simulink model "R4_ArduPilot_JSON"  (R2025b)
settings: Solver=ode4  StartTime=0.0  StopTime=P.stopTime  FixedStep=P.dt  RelTol=1e-3
InitFcn:
  | ww=get_param('R4_ArduPilot_JSON','ModelWorkspace'); pp=getVariable(ww,'P'); assignin(ww,'V',[pp.configurationCode(:);pp.mass(:);pp.cg(:);pp.inertia(:);pp.massCtrl(:);pp.cgCtrl(:);pp.inertiaCtrl(:);pp.g(:);pp.dt(:);pp.Ts(:);pp.stopTime(:);pp.sensorDelaySamples(:);pp.seed(:);pp.noiseScale(:);pp.sensorStd(:);pp.jetRadius(:);pp.motorRadius(:);pp.jetArea(:);pp.vaneArea(:);pp.vaneRadius(:);pp.forceZ(:);pp.hingeZ(:);pp.Lctrl(:);pp.CLalpha(:);pp.CLalphaCtrl(:);pp.stallAngle(:);pp.stallAngleCtrl(:);pp.effectiveness(:);pp.effectivenessCtrl(:);pp.CD0(:);pp.inducedDragK(:);pp.deltaMax(:);pp.servoRate(:);pp.servoTau(:);pp.fanTau(:);pp.fanTauCtrl(:);pp.TmaxNominal(:);pp.thrustScale(:);pp.voltageFinalScale(:);pp.voltageStart(:);pp.voltageRamp(:);pp.residualTorquePerN(:);pp.residualTorqueCtrl(:);pp.angularDrag(:);pp.linearDrag(:);pp.quadraticDrag(:);pp.angleGain(:);pp.rateKp(:);pp.rateKi(:);pp.rateLimit(:);pp.torqueIlimit(:);pp.altKp(:);pp.altKd(:);pp.altKi(:);pp.forceIlimit(:);pp.positionEnabled(:);pp.positionKp(:);pp.positionKd(:);pp.positionTiltLimit(:);pp.awTorque(:);pp.awForce(:);pp.controlEnabled(:);pp.scenario(:);pp.zReference(:);pp.initialEuler(:);pp.initialPosition(:);pp.initialVelocity(:);pp.forceDisturbance(:);pp.torqueDisturbance(:);pp.pulseTimes(:);pp.tetherEnabled(:);pp.groundEnabled(:);pp.tetherStiffness(:);pp.tetherDamping(:);pp.upperLength(:);pp.lowerLength(:);pp.groundStiffness(:);pp.groundDamping(:);pp.groundFriction(:);pp.controllerVersion(:);pp.heightPositionKp(:);pp.verticalSpeedKp(:);pp.verticalSpeedKi(:);pp.verticalSpeedLimit(:);pp.verticalAccelLimit(:);pp.throttleExpo(:);pp.startupEnabled(:);pp.startupSpoolBegin(:);pp.startupSpoolEnd(:);pp.startupRampNps(:);pp.startupMaxThrustFactor(:);pp.startupTimeout(:);pp.liftDetectHeight(:);pp.liftDetectDuration(:);pp.startupAbortTilt(:);pp.referenceGovernor(:);pp.tetherHeightLimit(:);pp.referenceStart(:);pp.referenceRiseTime(:);pp.referenceAngleStep(:);pp.referenceStepBegin(:);pp.referenceStepEnd(:);pp.staticTrimEnabled(:);pp.accelerationFilterTau(:);pp.eyeBody(:);pp.upperAnchor(:);pp.lowerAnchor(:);pp.feetBody(:);pp.floorZ(:);pp.trimT(:);pp.trimTau(:);pp.trimDelta(:);pp.x0(:);pp.y0(:);pp.trimWrench(:);pp.linkTs(:);pp.rangeNoiseStd(:);pp.rangeBias(:);pp.rangeSensorBodyZ(:);pp.rngSeed(:);pp.windWorld(:);pp.jsonPort(:)]); clear ww pp;
model workspace (MAT data in the model file):
  P.configurationCode = 5
  P.mass = 2.0128
  P.cg = [-0.00056; 0.00028; 0.31804]
  P.inertia = [0.042126; 0.042115; 0.007025]
  P.massCtrl = 2.0128
  P.cgCtrl = [-0.00056; 0.00028; 0.31804]
  P.inertiaCtrl = [0.042126; 0.042115; 0.007025]
  P.g = 9.80665
  P.dt = 0.000416666666667
  P.Ts = 0.005
  P.stopTime = 300
  P.sensorDelaySamples = 2
  P.seed = 41
  P.noiseScale = 1
  P.sensorStd = [0.001; 0.001; 0.001; 0.005; 0.005; 0.005; 0.00174532925199; 0.00174532925199; 0.00174532925199; 0.00349065850399; 0.00349065850399; 0.00349065850399; 0.05]
  P.jetRadius = 0.04
  P.motorRadius = 0.016
  P.jetArea = 0.00422230052642
  P.vaneArea = 0.000576
  P.vaneRadius = 0.031
  P.forceZ = 0.1316
  P.hingeZ = 0.13
  P.Lctrl = 0.18644
  P.CLalpha = 1.3
  P.CLalphaCtrl = 1.3
  P.stallAngle = 0.436332312999
  P.stallAngleCtrl = 0.436332312999
  P.effectiveness = 1
  P.effectivenessCtrl = 1
  P.CD0 = 0.015
  P.inducedDragK = 0.707355302631
  P.deltaMax = 0.349065850399
  P.servoRate = 12.3199711905
  P.servoTau = 0.03
  P.fanTau = 0.15
  P.fanTauCtrl = 0.15
  P.TmaxNominal = 27.6155264
  P.thrustScale = 1
  P.voltageFinalScale = 1
  P.voltageStart = 6
  P.voltageRamp = 1
  P.residualTorquePerN = 0.001
  P.residualTorqueCtrl = 0.001
  P.angularDrag = [0.002; 0.002; 0.001]
  P.linearDrag = [0.15; 0.15; 0.08]
  P.quadraticDrag = [0.08; 0.08; 0.05]
  P.angleGain = [2; 2; 1.8]
  P.rateKp = [0.32; 0.32; 0.08]
  P.rateKi = [0.35; 0.35; 0.08]
  P.rateLimit = [0.7; 0.7; 0.8]
  P.torqueIlimit = [0.15; 0.15; 0.06]
  P.altKp = 4
  P.altKd = 3.5
  P.altKi = 3
  P.forceIlimit = 8
  P.positionEnabled = 0
  P.positionKp = 0.6
  P.positionKd = 1.4
  P.positionTiltLimit = 0.13962634016
  P.awTorque = 6
  P.awForce = 2
  P.controlEnabled = 1
  P.scenario = 1
  P.zReference = 5
  P.initialEuler = [0; 0; 0]
  P.initialPosition = [0; 0; 0]
  P.initialVelocity = [0; 0; 0]
  P.forceDisturbance = [0  0; 0  0; 0  0]
  P.torqueDisturbance = [0  0; 0  0; 0  0]
  P.pulseTimes = [95  95.2; 105  105.5]
  P.tetherEnabled = 0
  P.groundEnabled = 1
  P.tetherStiffness = 5000
  P.tetherDamping = 35
  P.upperLength = 0.424
  P.lowerLength = 0.575
  P.groundStiffness = 8000
  P.groundDamping = 50
  P.groundFriction = 0.4
  P.controllerVersion = 2
  P.heightPositionKp = 1.2
  P.verticalSpeedKp = 6
  P.verticalSpeedKi = 2.5
  P.verticalSpeedLimit = 0.15
  P.verticalAccelLimit = 3
  P.throttleExpo = 0.6
  P.startupEnabled = 1
  P.startupSpoolBegin = 0.5
  P.startupSpoolEnd = 2
  P.startupRampNps = 1.2
  P.startupMaxThrustFactor = 1.32
  P.startupTimeout = 14
  P.liftDetectHeight = 0.008
  P.liftDetectDuration = 0.05
  P.startupAbortTilt = 0.349065850399
  P.referenceGovernor = 1
  P.tetherHeightLimit = 0.075
  P.referenceStart = 2
  P.referenceRiseTime = 4
  P.referenceAngleStep = [0; 0; 0]
  P.referenceStepBegin = 9
  P.referenceStepEnd = 12
  P.staticTrimEnabled = 1
  P.accelerationFilterTau = 0.1
  P.eyeBody = [0.0698564645563  -0.0687364645563  -0.0687364645563  0.0698564645563; 0.0690164645563  0.0690164645563  -0.0695764645563  -0.0695764645563; 0.11946  0.11946  0.11946  0.11946]
  P.upperAnchor = [0.270674790413  -0.269554790413  -0.269554790413  0.270674790413; 0.269834790413  0.269834790413  -0.270394790413  -0.270394790413; 0.43396  0.43396  0.43396  0.43396]
  P.lowerAnchor = [0.25056  -0.24944  -0.24944  0.25056; 0.16472  0.16472  -0.16528  -0.16528; -0.31804  -0.31804  -0.31804  -0.31804]
  P.feetBody = [0.163194559673  -0.162074559673  -0.162074559673  0.163194559673; 0.162354559673  0.162354559673  -0.162914559673  -0.162914559673; -0.33304  -0.33304  -0.33304  -0.33304]
  P.floorZ = -0.33304
  P.trimT = 19.8749456665
  P.trimTau = [0.00556498478663; 0.0111299695733; -0.0198749456665]
  P.trimDelta = [-0.0825320279718; -0.0740418704167; -0.099550958918; -0.108087721792]
  P.x0 = [0; 0; 0; 0; 0; 0; 1; 0; 0; 0; 0; 0; 0; 0; 0; 0; 0; 0]
  P.y0 = [0; 0; 0; 0; 0; 0; 0; 0; 0; 0; 0; 0; 0]
  P.trimWrench = [19.8749456665; 0.00556498478663; 0.0111299695733; -0.0198749456665]
  P.linkTs = 0.000833333333333
  P.rangeNoiseStd = 0.02
  P.rangeBias = 0
  P.rangeSensorBodyZ = -0.20304
  P.rngSeed = 2107
  P.windWorld = [1; 0; 0]
  P.jsonPort = 9002
  V = [5; 2.0128; -0.00056; 0.00028; 0.31804; 0.042126; 0.042115; 0.007025; 2.0128; -0.00056; 0.00028; 0.31804; 0.042126; 0.042115; 0.007025; 9.80665; 0.000416666666667; 0.005; 300; 2; 41; 1; 0.001; 0.001; 0.001; 0.005; 0.005; 0.005; 0.00174532925199; 0.00174532925199; 0.00174532925199; 0.00349065850399; 0.00349065850399; 0.00349065850399; 0.05; 0.04; 0.016; 0.00422230052642; 0.000576; 0.031; 0.1316; 0.13; 0.18644; 1.3; 1.3; 0.436332312999; 0.436332312999; 1; 1; 0.015; 0.707355302631; 0.349065850399; 12.3199711905; 0.03; 0.15; 0.15; 27.6155264; 1; 1; 6; 1; 0.001; 0.001; 0.002; 0.002; 0.001; 0.15; 0.15; 0.08; 0.08; 0.08; 0.05; 2; 2; 1.8; 0.32; 0.32; 0.08; 0.35; 0.35; 0.08; 0.7; 0.7; 0.8; 0.15; 0.15; 0.06; 4; 3.5; 3; 8; 0; 0.6; 1.4; 0.13962634016; 6; 2; 1; 1; 5; 0; 0; 0; 0; 0; 0; 0; 0; 0; 0; 0; 0; 0; 0; 0; 0; 0; 0; 0; 0; 0; 95; 105; 95.2; 105.5; 0; 1; 5000; 35; 0.424; 0.575; 8000; 50; 0.4; 2; 1.2; 6; 2.5; 0.15; 3; 0.6; 1; 0.5; 2; 1.2; 1.32; 14; 0.008; 0.05; 0.349065850399; 1; 0.075; 2; 4; 0; 0; 0; 9; 12; 1; 0.1; 0.0698564645563; 0.0690164645563; 0.11946; -0.0687364645563; 0.0690164645563; 0.11946; -0.0687364645563; -0.0695764645563; 0.11946; 0.0698564645563; -0.0695764645563; 0.11946; 0.270674790413; 0.269834790413; 0.43396; -0.269554790413; 0.269834790413; 0.43396; -0.269554790413; -0.270394790413; 0.43396; 0.270674790413; -0.270394790413; 0.43396; 0.25056; 0.16472; -0.31804; -0.24944; 0.16472; -0.31804; -0.24944; -0.16528; -0.31804; 0.25056; -0.16528; -0.31804; 0.163194559673; 0.162354559673; -0.33304; -0.162074559673; 0.162354559673; -0.33304; -0.162074559673; -0.162914559673; -0.33304; 0.163194559673; -0.162914559673; -0.33304; -0.33304; 19.8749456665; 0.00556498478663; 0.0111299695733; -0.0198749456665; -0.0825320279718; -0.0740418704167; -0.099550958918; -0.108087721792; 0; 0; 0; 0; 0; 0; 1; 0; 0; 0; 0; 0; 0; 0; 0; 0; 0; 0; 0; 0; 0; 0; 0; 0; 0; 0; 0; 0; 0; 0; 0; 19.8749456665; 0.00556498478663; 0.0111299695733; -0.0198749456665; 0.000833333333333; 0.02; 0; -0.20304; 2107; 1; 0; 0; 9002]
values from neighbouring files (symbols this model uses):
  P = jsondecode(fileread(fullfile(folder,'design_parameters.json')))    [ap_parameters.m]    (also in r4_ap_send.m = R4_AP_PARAMETERS; run_ap_case.m = ap_parameters(name))
settings Model: Creator=izais  LastModifiedBy=izais
settings DataIOCC: SaveOutput=off  SignalLogging=off  SaveTime=off
settings DebuggingCC: AlgebraicLoopMsg=error

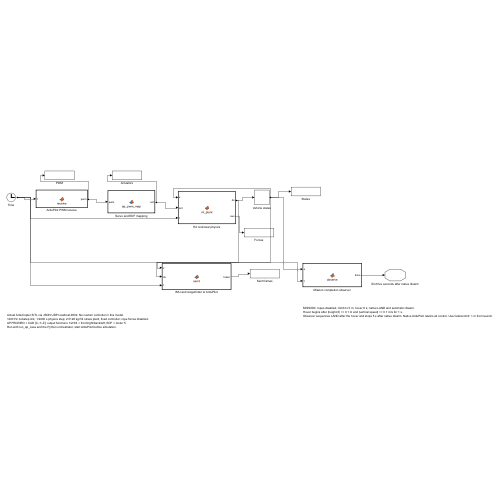
[thumbnail: Simulink's stored preview of the top-level diagram]
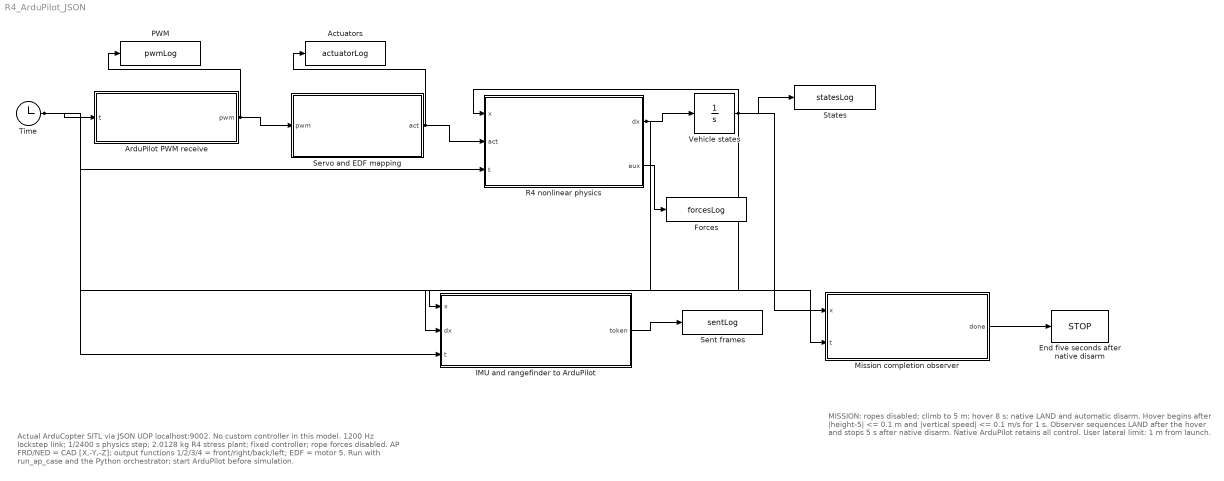
== system R4_ArduPilot_JSON ==
  note: Actual ArduCopter SITL via JSON UDP localhost:9002. No custom controller in this model.
      | 1200 Hz lockstep link; 1/2400 s physics step; 2.0128 kg R4 stress plant; fixed controller; rope forces disabled.
      | AP FRD/NED = CAD [X,-Y,-Z]; output functions 1/2/3/4 = front/right/back/left; EDF = motor 5.
      | Run with run_ap_case and the Python orchestrator; start ArduPilot before simulation.
  note: MISSION: ropes disabled; climb to 5 m; hover 8 s; native LAND and automatic disarm.
      | Hover begins after |height-5| <= 0.1 m and |vertical speed| <= 0.1 m/s for 1 s.
      | Observer sequences LAND after the hover and stops 5 s after native disarm. Native ArduPilot retains all control. User lateral limit: 1 m from launch.
  Actuators : ToWorkspace  VariableName=actuatorLog  SaveFormat=Timeseries  SampleTime=P.linkTs
  ArduPilot PWM receive : MATLAB Function  TreatAsAtomicUnit=on
  End five seconds after native disarm : Stop
  Forces : ToWorkspace  VariableName=forcesLog  SaveFormat=Timeseries  SampleTime=P.linkTs
  IMU and rangefinder to ArduPilot : MATLAB Function  TreatAsAtomicUnit=on
  Mission completion observer : MATLAB Function  TreatAsAtomicUnit=on
  PWM : ToWorkspace  VariableName=pwmLog  SaveFormat=Timeseries  SampleTime=P.linkTs
  R4 nonlinear physics : MATLAB Function  TreatAsAtomicUnit=on
  Sent frames : ToWorkspace  VariableName=sentLog  SaveFormat=Timeseries  SampleTime=P.linkTs
  Servo and EDF mapping : MATLAB Function  TreatAsAtomicUnit=on
  States : ToWorkspace  VariableName=statesLog  SaveFormat=Timeseries  SampleTime=P.linkTs
  Time : Clock
  Vehicle states : Integrator  InitialCondition=P.x0
  wires:
  Time/1 -> ArduPilot PWM receive/1(t), R4 nonlinear physics/3(t), IMU and rangefinder to ArduPilot/3(t), Mission completion observer/2(t)
  ArduPilot PWM receive/1(pwm) -> Servo and EDF mapping/1(pwm), PWM/1
  Servo and EDF mapping/1(act) -> R4 nonlinear physics/2(act), Actuators/1
  R4 nonlinear physics/1(dx) -> Vehicle states/1, IMU and rangefinder to ArduPilot/2(dx)
  Vehicle states/1 -> R4 nonlinear physics/1(x), IMU and rangefinder to ArduPilot/1(x), States/1, Mission completion observer/1(x)
  R4 nonlinear physics/2(aux) -> Forces/1
  IMU and rangefinder to ArduPilot/1(token) -> Sent frames/1
  Mission completion observer/1(done) -> End five seconds after native disarm/1

== matlab function R4_ArduPilot_JSON/Servo and EDF mapping ==
  data: pwm input; act output; V parameter
function act=ap_pwm_map(pwm, V)
P.configurationCode=V(1);
P.mass=V(2);
P.cg=reshape(V(3:5),3,1);
P.inertia=reshape(V(6:8),3,1);
P.massCtrl=V(9);
P.cgCtrl=reshape(V(10:12),3,1);
P.inertiaCtrl=reshape(V(13:15),3,1);
P.g=V(16);
P.dt=V(17);
P.Ts=V(18);
P.stopTime=V(19);
P.sensorDelaySamples=V(20);
P.seed=V(21);
P.noiseScale=V(22);
P.sensorStd=reshape(V(23:35),13,1);
P.jetRadius=V(36);
P.motorRadius=V(37);
P.jetArea=V(38);
P.vaneArea=V(39);
P.vaneRadius=V(40);
P.forceZ=V(41);
P.hingeZ=V(42);
P.Lctrl=V(43);
P.CLalpha=V(44);
P.CLalphaCtrl=V(45);
P.stallAngle=V(46);
P.stallAngleCtrl=V(47);
P.effectiveness=V(48);
P.effectivenessCtrl=V(49);
P.CD0=V(50);
P.inducedDragK=V(51);
P.deltaMax=V(52);
P.servoRate=V(53);
P.servoTau=V(54);
P.fanTau=V(55);
P.fanTauCtrl=V(56);
P.TmaxNominal=V(57);
P.thrustScale=V(58);
P.voltageFinalScale=V(59);
P.voltageStart=V(60);
P.voltageRamp=V(61);
P.residualTorquePerN=V(62);
P.residualTorqueCtrl=V(63);
P.angularDrag=reshape(V(64:66),3,1);
P.linearDrag=reshape(V(67:69),3,1);
P.quadraticDrag=reshape(V(70:72),3,1);
P.angleGain=reshape(V(73:75),3,1);
P.rateKp=reshape(V(76:78),3,1);
P.rateKi=reshape(V(79:81),3,1);
P.rateLimit=reshape(V(82:84),3,1);
P.torqueIlimit=reshape(V(85:87),3,1);
P.altKp=V(88);
P.altKd=V(89);
P.altKi=V(90);
P.forceIlimit=V(91);
P.positionEnabled=V(92);
P.positionKp=V(93);
P.positionKd=V(94);
P.positionTiltLimit=V(95);
P.awTorque=V(96);
P.awForce=V(97);
P.controlEnabled=V(98);
P.scenario=V(99);
P.zReference=V(100);
P.initialEuler=reshape(V(101:103),3,1);
P.initialPosition=reshape(V(104:106),3,1);
P.initialVelocity=reshape(V(107:109),3,1);
P.forceDisturbance=reshape(V(110:115),3,2);
P.torqueDisturbance=reshape(V(116:121),3,2);
P.pulseTimes=reshape(V(122:125),2,2);
P.tetherEnabled=V(126);
P.groundEnabled=V(127);
P.tetherStiffness=V(128);
P.tetherDamping=V(129);
P.upperLength=V(130);
P.lowerLength=V(131);
P.groundStiffness=V(132);
P.groundDamping=V(133);
P.groundFriction=V(134);
P.controllerVersion=V(135);
P.heightPositionKp=V(136);
P.verticalSpeedKp=V(137);
P.verticalSpeedKi=V(138);
P.verticalSpeedLimit=V(139);
P.verticalAccelLimit=V(140);
P.throttleExpo=V(141);
P.startupEnabled=V(142);
P.startupSpoolBegin=V(143);
P.startupSpoolEnd=V(144);
P.startupRampNps=V(145);
P.startupMaxThrustFactor=V(146);
P.startupTimeout=V(147);
P.liftDetectHeight=V(148);
P.liftDetectDuration=V(149);
P.startupAbortTilt=V(150);
P.referenceGovernor=V(151);
P.tetherHeightLimit=V(152);
P.referenceStart=V(153);
P.referenceRiseTime=V(154);
P.referenceAngleStep=reshape(V(155:157),3,1);
P.referenceStepBegin=V(158);
P.referenceStepEnd=V(159);
P.staticTrimEnabled=V(160);
P.accelerationFilterTau=V(161);
P.eyeBody=reshape(V(162:173),3,4);
P.upperAnchor=reshape(V(174:185),3,4);
P.lowerAnchor=reshape(V(186:197),3,4);
P.feetBody=reshape(V(198:209),3,4);
P.floorZ=V(210);
P.trimT=V(211);
P.trimTau=reshape(V(212:214),3,1);
P.trimDelta=reshape(V(215:218),4,1);
P.x0=reshape(V(219:236),18,1);
P.y0=reshape(V(237:249),13,1);
P.trimWrench=reshape(V(250:253),4,1);
P.linkTs=V(254);
P.rangeNoiseStd=V(255);
P.rangeBias=V(256);
P.rangeSensorBodyZ=V(257);
P.rngSeed=V(258);
P.windWorld=reshape(V(259:261),3,1);
P.jsonPort=V(262);

% AP FRD axes correspond to CAD [X,-Y,-Z]. Front/right/back/left vanes
% are CAD +X/-Y/-X/+Y. Physical positive deflection is CAD tangent +phi.
act=zeros(5,1);act(1)=max(0,min(1,(pwm(5)-1000)/1000));
channel=[1,4,3,2];
for k=1:4
    value=pwm(channel(k));
    if value<900,value=1500;end % no valid pulse during firmware initialization
    act(k+1)=max(-1,min(1,(value-1500)/500))*P.deltaMax;
end
end

== matlab function R4_ArduPilot_JSON/ArduPilot PWM receive ==
  settings: updateMethod=DISCRETE  sampleTime=P.linkTs
  data: t input; pwm output
function pwm=receive(t)
coder.extrinsic('r4_ap_receive');
pwm=zeros(16,1);pwm=r4_ap_receive(t);
end

== matlab function R4_ArduPilot_JSON/R4 nonlinear physics ==
  data: x input; dx output; act input; t input; aux output; V parameter
function [dx, aux] = r4_plant(x, act, t, V)
P.configurationCode=V(1);
P.mass=V(2);
P.cg=reshape(V(3:5),3,1);
P.inertia=reshape(V(6:8),3,1);
P.massCtrl=V(9);
P.cgCtrl=reshape(V(10:12),3,1);
P.inertiaCtrl=reshape(V(13:15),3,1);
P.g=V(16);
P.dt=V(17);
P.Ts=V(18);
P.stopTime=V(19);
P.sensorDelaySamples=V(20);
P.seed=V(21);
P.noiseScale=V(22);
P.sensorStd=reshape(V(23:35),13,1);
P.jetRadius=V(36);
P.motorRadius=V(37);
P.jetArea=V(38);
P.vaneArea=V(39);
P.vaneRadius=V(40);
P.forceZ=V(41);
P.hingeZ=V(42);
P.Lctrl=V(43);
P.CLalpha=V(44);
P.CLalphaCtrl=V(45);
P.stallAngle=V(46);
P.stallAngleCtrl=V(47);
P.effectiveness=V(48);
P.effectivenessCtrl=V(49);
P.CD0=V(50);
P.inducedDragK=V(51);
P.deltaMax=V(52);
P.servoRate=V(53);
P.servoTau=V(54);
P.fanTau=V(55);
P.fanTauCtrl=V(56);
P.TmaxNominal=V(57);
P.thrustScale=V(58);
P.voltageFinalScale=V(59);
P.voltageStart=V(60);
P.voltageRamp=V(61);
P.residualTorquePerN=V(62);
P.residualTorqueCtrl=V(63);
P.angularDrag=reshape(V(64:66),3,1);
P.linearDrag=reshape(V(67:69),3,1);
P.quadraticDrag=reshape(V(70:72),3,1);
P.angleGain=reshape(V(73:75),3,1);
P.rateKp=reshape(V(76:78),3,1);
P.rateKi=reshape(V(79:81),3,1);
P.rateLimit=reshape(V(82:84),3,1);
P.torqueIlimit=reshape(V(85:87),3,1);
P.altKp=V(88);
P.altKd=V(89);
P.altKi=V(90);
P.forceIlimit=V(91);
P.positionEnabled=V(92);
P.positionKp=V(93);
P.positionKd=V(94);
P.positionTiltLimit=V(95);
P.awTorque=V(96);
P.awForce=V(97);
P.controlEnabled=V(98);
P.scenario=V(99);
P.zReference=V(100);
P.initialEuler=reshape(V(101:103),3,1);
P.initialPosition=reshape(V(104:106),3,1);
P.initialVelocity=reshape(V(107:109),3,1);
P.forceDisturbance=reshape(V(110:115),3,2);
P.torqueDisturbance=reshape(V(116:121),3,2);
P.pulseTimes=reshape(V(122:125),2,2);
P.tetherEnabled=V(126);
P.groundEnabled=V(127);
P.tetherStiffness=V(128);
P.tetherDamping=V(129);
P.upperLength=V(130);
P.lowerLength=V(131);
P.groundStiffness=V(132);
P.groundDamping=V(133);
P.groundFriction=V(134);
P.controllerVersion=V(135);
P.heightPositionKp=V(136);
P.verticalSpeedKp=V(137);
P.verticalSpeedKi=V(138);
P.verticalSpeedLimit=V(139);
P.verticalAccelLimit=V(140);
P.throttleExpo=V(141);
P.startupEnabled=V(142);
P.startupSpoolBegin=V(143);
P.startupSpoolEnd=V(144);
P.startupRampNps=V(145);
P.startupMaxThrustFactor=V(146);
P.startupTimeout=V(147);
P.liftDetectHeight=V(148);
P.liftDetectDuration=V(149);
P.startupAbortTilt=V(150);
P.referenceGovernor=V(151);
P.tetherHeightLimit=V(152);
P.referenceStart=V(153);
P.referenceRiseTime=V(154);
P.referenceAngleStep=reshape(V(155:157),3,1);
P.referenceStepBegin=V(158);
P.referenceStepEnd=V(159);
P.staticTrimEnabled=V(160);
P.accelerationFilterTau=V(161);
P.eyeBody=reshape(V(162:173),3,4);
P.upperAnchor=reshape(V(174:185),3,4);
P.lowerAnchor=reshape(V(186:197),3,4);
P.feetBody=reshape(V(198:209),3,4);
P.floorZ=V(210);
P.trimT=V(211);
P.trimTau=reshape(V(212:214),3,1);
P.trimDelta=reshape(V(215:218),4,1);
P.x0=reshape(V(219:236),18,1);
P.y0=reshape(V(237:249),13,1);
P.trimWrench=reshape(V(250:253),4,1);
P.linkTs=V(254);
P.rangeNoiseStd=V(255);
P.rangeBias=V(256);
P.rangeSensorBodyZ=V(257);
P.rngSeed=V(258);
P.windWorld=reshape(V(259:261),3,1);
P.jsonPort=V(262);

% Nonlinear six-degree-of-freedom rigid body, quaternion attitude, fan and
% servo dynamics. CAD X/Y are transverse; CAD +Z is upward thrust.
pos=x(1:3);vel=x(4:6);q=x(7:10);qn=q/max(norm(q),1e-12);
w=qn(1);a=qn(2);b=qn(3);c=qn(4);
R=[1-2*(b*b+c*c),2*(a*b-w*c),2*(a*c+w*b);...
   2*(a*b+w*c),1-2*(a*a+c*c),2*(b*c-w*a);...
   2*(a*c-w*b),2*(b*c+w*a),1-2*(a*a+b*b)];
omega=x(11:13);T=max(0,x(14));delta=max(-P.deltaMax,min(P.deltaMax,x(15:18)));
v=1+(P.voltageFinalScale-1)*max(0,min(1,(t-P.voltageStart)/max(P.voltageRamp,0.01)));
Tmax=P.TmaxNominal*P.thrustScale*v;
throttle=max(0,min(1,act(1)));
Ttarget=Tmax*((1-P.throttleExpo)*throttle+P.throttleExpo*throttle^2);
dT=(Ttarget-x(14))/P.fanTau;
deltaTarget=max(-P.deltaMax,min(P.deltaMax,act(2:5)));
ddelta=max(-P.servoRate,min(P.servoRate,(deltaTarget-x(15:18))/P.servoTau));
cl=P.CLalpha*delta./sqrt(1+(delta/P.stallAngle).^4);
qS=T/(2*P.jetArea)*P.vaneArea*P.effectiveness;
fv=qS*cl;drag=qS*(P.CD0+P.inducedDragK*cl.^2);
forceBody=[0;0;T];tau=cross([-P.cg(1);-P.cg(2);0],[0;0;T]);
for k=1:4
    phi=(k-1)*pi/2;tanvec=[-sin(phi);cos(phi);0];
    ff=tanvec*fv(k)+[0;0;-drag(k)];
    arm=[P.vaneRadius*cos(phi);P.vaneRadius*sin(phi);P.forceZ]-P.cg;
    forceBody=forceBody+ff;tau=tau+cross(arm,ff);
end
tau=tau+[0;0;P.residualTorquePerN*T]-P.angularDrag.*omega;
airVelocity=vel-P.windWorld;
forceWorld=R*forceBody-[0;0;P.mass*P.g]-P.linearDrag.*airVelocity-P.quadraticDrag.*abs(airVelocity).*airVelocity;
for n=1:2
    if t>=P.pulseTimes(n,1) && t<P.pulseTimes(n,2)
        forceWorld=forceWorld+P.forceDisturbance(:,n);tau=tau+P.torqueDisturbance(:,n);
    end
end
maxTension=0;ropeForce=zeros(3,1);groundForce=0;
if P.tetherEnabled>0.5
    for k=1:4
        rb=P.eyeBody(:,k);eye=pos+R*rb;eyeVelocity=vel+R*cross(omega,rb);
        for j=1:2
            if j==1,anchor=P.upperAnchor(:,k);L=P.upperLength;
            else,anchor=P.lowerAnchor(:,k);L=P.lowerLength;end
            diff=anchor-eye;d=norm(diff);dir=diff/max(d,1e-12);excess=d-L;
            if excess>0
                extensionRate=-dot(eyeVelocity,dir);
                tension=max(0,P.tetherStiffness*excess+P.tetherDamping*extensionRate);
                ff=tension*dir;forceWorld=forceWorld+ff;ropeForce=ropeForce+ff;
                tau=tau+cross(rb,R'*ff);maxTension=max(maxTension,tension);
            end
        end
    end
end
if P.groundEnabled>0.5
    for k=1:4
        rb=P.feetBody(:,k);foot=pos+R*rb;vv=vel+R*cross(omega,rb);
        if foot(3)<P.floorZ
            fn=max(0,P.groundStiffness*(P.floorZ-foot(3))-P.groundDamping*vv(3));
            ft=-P.groundFriction*fn*tanh(vv(1:2)/0.03);ff=[ft;fn];
            forceWorld=forceWorld+ff;tau=tau+cross(rb,R'*ff);groundForce=groundForce+fn;
        end
    end
end
pp=omega(1);qq=omega(2);rr=omega(3);
Q=[0,-pp,-qq,-rr;pp,0,rr,-qq;qq,-rr,0,pp;rr,qq,-pp,0];
dq=0.5*Q*q+0.5*(1-dot(q,q))*q;
angularAcceleration=(tau-cross(omega,P.inertia.*omega))./P.inertia;
dx=[vel;forceWorld/P.mass;dq;angularAcceleration;dT;ddelta];
cllim=P.CLalpha*P.deltaMax/sqrt(1+(P.deltaMax/P.stallAngle)^4);
spinMargin=4*P.vaneRadius*qS*cllim-abs(P.residualTorquePerN*T);
aux=[fv;forceBody(3);sum(drag);Tmax;maxTension;groundForce;tau;norm(ropeForce);...
     spinMargin;norm(q)-1;P.mass*P.g];
end

== matlab function R4_ArduPilot_JSON/IMU and rangefinder to ArduPilot ==
  settings: updateMethod=DISCRETE  sampleTime=P.linkTs
  data: x input; token output; dx input; t input
function token=send(x,dx,t)
coder.extrinsic('r4_ap_send');
r4_ap_send(x,dx,t);token=t;
end

== matlab function R4_ArduPilot_JSON/Mission completion observer ==
  settings: updateMethod=DISCRETE  sampleTime=0.0008333333333333334
  data: x input; done output; t input
function done=observe(x,t)
coder.extrinsic('r4_mission_supervise');
done=false;done=r4_mission_supervise(x,t);
end
